simulink model "fix_Current_sync"  (R2025b)
settings: Solver=FixedStepAuto  StartTime=0.0  StopTime=20  FixedStep=0.001  RelTol=1e-3
values from neighbouring files (symbols this model uses):
  Dm = 1e-3    (= 0.001)    [motor_param.m]
  Ki_s = 0.041    [motor_param.m]
  Kp_s = 0.0014    [motor_param.m]
  Ld = 0.01    [motor_param.m]
  Lq = 0.02    [motor_param.m]
  p = 2    [motor_param.m]
  Phi = 0.1    [motor_param.m]
  Rs = 0.38    [motor_param.m]
libraries: fl_lib x50, nesl_utility x50, ee_lib x15, eeTransforms x10, slpidlib x5
(part 3 of 3)

== system fix_Current_sync/Subsystem5/Plant/MechSensor ==
  Ideal Rotational Motion Sensor : fl_lib/Mechanical/Mechanical Sensors/Ideal Rotational Motion Sensor  reference=foundation.enum.MeasurementReference.difference  acceleration_port=false  velocity_port=true  position_port=true  wrap_angle=simscape.enum.onoff.off  offset=0 rad
  Ideal Torque Sensor : fl_lib/Mechanical/Mechanical Sensors/Ideal Torque Sensor
  PS-Simulink Converter : nesl_utility/PS-Simulink Converter  PhysicalDomain=network_engine_domain  SubClassName=ps_output  LeftPortType=input  RightPortType=output  PseudoPeriodic=off  Frequencies=[]  VectorFormat=1-D array  Unit=1  AffineConversion=off
  PS-Simulink Converter1 : nesl_utility/PS-Simulink Converter  PhysicalDomain=network_engine_domain  SubClassName=ps_output  LeftPortType=input  RightPortType=output  PseudoPeriodic=off  Frequencies=[]  VectorFormat=1-D array  Unit=1  AffineConversion=off
  PS-Simulink Converter2 : nesl_utility/PS-Simulink Converter  PhysicalDomain=network_engine_domain  SubClassName=ps_output  LeftPortType=input  RightPortType=output  PseudoPeriodic=off  Frequencies=[]  VectorFormat=1-D array  Unit=1  AffineConversion=off
  R1 : PMIOPort  Side=Left
  C1 : PMIOPort  Port=2  Side=Left
  R2 : PMIOPort  Port=3  Side=Right
  C2 : PMIOPort  Port=4  Side=Right
  wm : Outport  VectorParamsAs1DForOutWhenUnconnected=off
  thm : Outport  Port=2  VectorParamsAs1DForOutWhenUnconnected=off
  Tm : Outport  Port=3  VectorParamsAs1DForOutWhenUnconnected=off
  wires:
  PS-Simulink Converter/1 -> thm/1
  PS-Simulink Converter1/1 -> Tm/1
  PS-Simulink Converter2/1 -> wm/1
  connections:
  Ideal Rotational Motion Sensor/RConn3 -- PS-Simulink Converter/LConn1
  Ideal Rotational Motion Sensor/RConn1 -- C2/RConn1 -- C1/RConn1
  Ideal Torque Sensor/LConn1 -- R1/RConn1
  Ideal Torque Sensor/RConn1 -- R2/RConn1 -- Ideal Rotational Motion Sensor/LConn1
  PS-Simulink Converter1/LConn1 -- Ideal Torque Sensor/RConn2
  Ideal Rotational Motion Sensor/RConn2 -- PS-Simulink Converter2/LConn1

== system fix_Current_sync/Subsystem1/Controller/DriverPeripherals/Break Algebraic Loop ==
  In1 : Inport
  Demux : Demux  Outputs=3
  Mux : Mux  Inputs=3
  Transfer Fcn : TransferFcn  Denominator=[1e-6 1]
  Transfer Fcn1 : TransferFcn  Denominator=[1e-6 1]
  Transfer Fcn2 : TransferFcn  Denominator=[1e-6 1]
  Out1 : Outport
  wires:
  In1/1 -> Demux/1
  Demux/1 -> Transfer Fcn/1
  Transfer Fcn/1 -> Mux/1
  Demux/2 -> Transfer Fcn1/1
  Transfer Fcn1/1 -> Mux/2
  Demux/3 -> Transfer Fcn2/1
  Transfer Fcn2/1 -> Mux/3
  Mux/1 -> Out1/1

== system fix_Current_sync/Subsystem1/Controller/FOC/CurrentController ==
  Iqref : Inport
  Id : Inport  Port=2
  Iq : Inport  Port=3
  we : Inport  Port=4
  Integrator : Integrator
  MATLAB Function : MATLAB Function  TreatAsAtomicUnit=on
  Scope : Scope
      settings: ActiveDisplayYMinimum=-0.021972241997855933  ActiveDisplayYMaximum=0.011100987286103392  DataLoggingVariableName=ScopeData15
  Scope1 : Scope
      settings: ActiveDisplayYMinimum=-15.558960108709503  ActiveDisplayYMaximum=12.807301262932642  DataLoggingVariableName=ScopeData10
  Scope2 : Scope
      settings: ActiveDisplayYMinimum=-2.450488291060998  ActiveDisplayYMaximum=2.3822321131147937  DataLoggingVariableName=ScopeData11
  Vdref : Outport  VectorParamsAs1DForOutWhenUnconnected=off
  Vqref : Outport  Port=2  VectorParamsAs1DForOutWhenUnconnected=off
  wires:
  Integrator/1 -> MATLAB Function/1(z_q)
  MATLAB Function/3(dz_q) -> Integrator/1
  MATLAB Function/4(e_q_bar) -> Scope/1
  MATLAB Function/1(Vq) -> Scope1/1, Vqref/1
  MATLAB Function/2(Vd) -> Scope2/1, Vdref/1
  we/1 -> MATLAB Function/5(we)
  Iqref/1 -> MATLAB Function/2(i_q_ref)
  Id/1 -> MATLAB Function/4(i_d)
  Iq/1 -> MATLAB Function/3(i_q)

== system fix_Current_sync/Subsystem1/Controller/FOC/VelocityController ==
  wmref : Inport
  wm : Inport  Port=2
  Gain : Gain  Gain=1/(3/2*p*Phi)
  PIDController : slpidlib/PID Controller  Controller=PI  Form=Parallel  TimeDomain=Continuous-time  UseExternalTs=off  SampleTime=-1  IntegratorMethod=Forward Euler  FilterMethod=Forward Euler  ControllerParametersSource=internal  P=Kp_s  I=Ki_s  UseKiTs=off  D=0  UseExternalDerivativeSource=off  N=100  UseFilter=on  TunerSelectOption=Transfer Function Based (PID Tuner App)  InitialConditionSource=internal  InitialConditionForIntegrator=0  InitialConditionForFilter=0  DifferentiatorICPrevScaledInput=0  ExternalReset=none  TrackingMode=off  Kt=1  LimitOutput=off  SatLimitsSource=internal  UpperSaturationLimit=inf  LowerSaturationLimit=-inf  LinearizeAsGain=on  AntiWindupMode=none  Kb=1  LimitIntegrator=off  UpperIntegratorSaturationLimit=inf  LowerIntegratorSaturationLimit=-inf  POutMin=[]  POutMax=[]  IOutMin=[]  IOutMax=[]  DOutMin=[]  DOutMax=[]  NOutMin=[]  NOutMax=[]  SumOutMin=[]  SumOutMax=[]  SaturationOutMin=[]  SaturationOutMax=[]  PParamMin=[]  PParamMax=[]  IParamMin=[]  IParamMax=[]  DParamMin=[]  DParamMax=[]  NParamMin=[]  NParamMax=[]  KbParamMin=[]  KbParamMax=[]  KtParamMin=[]  KtParamMax=[]  KbOutMin=[]  KbOutMax=[]  KtOutMin=[]  KtOutMax=[]  IntegratorOutMin=[]  IntegratorOutMax=[]  FilterOutMin=[]  FilterOutMax=[]  SumI1OutMin=[]  SumI1OutMax=[]  SumI2OutMin=[]  SumI2OutMax=[]  SumI3OutMin=[]  SumI3OutMax=[]  SumI4OutMin=[]  SumI4OutMax=[]  SumDOutMin=[]  SumDOutMax=[]  DifferentiatorOutMin=[]  DifferentiatorOutMax=[]  FilterDiffOutCoefMin=[]  FilterDiffOutCoefMax=[]  ReciprocalOutMin=[]  ReciprocalOutMax=[]  SumDenOutMin=[]  SumDenOutMax=[]  SumNumOutMin=[]  SumNumOutMax=[]  DivideOutMin=[]  DivideOutMax=[]  UdiffTsProdOutMin=[]  UdiffTsProdOutMax=[]  NTsProdOutMin=[]  NTsProdOutMax=[]  UintegralTsProdOutMin=[]  UintegralTsProdOutMax=[]  UngainTsProdOutMin=[]  UngainTsProdOutMax=[]  ClampingZeroOutDataTypeStr=Inherit: Inherit via back propagation  ClampingZeroOutMin=[]  ClampingZeroOutMax=[]  FilterDenConstantOutDataTypeStr=Inherit: Inherit via back propagation  FilterDenConstantOutMin=[]  FilterDenConstantOutMax=[]  PCopyOutDataTypeStr=Inherit: Inherit via back propagation  PCopyOutMin=[]  PCopyOutMax=[]  NCopyOutDataTypeStr=Inherit: Inherit via back propagation  NCopyOutMin=[]  NCopyOutMax=[]  IntegratorContinuousStateAttributes=''  IntegratorStateMustResolveToSignalObject=off  IntegratorRTWStateStorageClass=Auto  FilterContinuousStateAttributes=''  FilterStateMustResolveToSignalObject=off  FilterRTWStateStorageClass=Auto  ParallelPVariant=InternalParameters  IdealPVariant=Disabled  IVariant=InternalParameters  DVariant=Disabled  IntegratorVariant=Continuous  SatVariant=Disabled  AWVariant=Passthrough  PCopyVariant=Disabled  TRVariant=Disabled  FdbkBlocksVariant=Forward  IdealPFdbkVariant=Disabled  SatFdbkVariant=Disabled  DerivativeFilterVariant=Disabled  NVariant=Disabled  NCopyVariant=Disabled_SignalSpec  FilterICVariant=Disabled  IntegratorICVariant=InternalICs  ExternalResetVariant=Disabled  TRSumVariant=Passthrough  SumFdbkVariant=Disabled  SumVariant=Sum_PI  TsampFilterVariant=InternalTs  TsampNgainVariant=Passthrough  TsampIntegralVariant=Disabled_SignalSpec  ExternalSaturationOutDataTypeStr=Inherit: Same as second input  DerivativeSourceVariant=Disabled  PreIntVariant=InternalPreInt
  Sum : Sum  Inputs=|+-
  Iqref : Outport  VectorParamsAs1DForOutWhenUnconnected=off
  wires:
  Gain/1 -> Iqref/1
  wmref/1 -> Sum/1
  wm/1 -> Sum/2
  Sum/1 -> PIDController/1
  PIDController/1 -> Gain/1

== system fix_Current_sync/Subsystem1/Controller/FOC/abc2dq ==
  Iabc : Inport
  thetae : Inport  Port=2
  Demux1 : Demux  Outputs=3
  Park Transform : eeTransforms/Park Transform  AxisAlignment=D-axis  PowerInvariant=off
  Terminator : Terminator
  Id : Outport  VectorParamsAs1DForOutWhenUnconnected=off
  Iq : Outport  Port=2  VectorParamsAs1DForOutWhenUnconnected=off
  wires:
  Iabc/1 -> Park Transform/1
  thetae/1 -> Park Transform/2
  Demux1/3 -> Terminator/1
  Park Transform/1 -> Demux1/1
  Demux1/1 -> Id/1
  Demux1/2 -> Iq/1

== system fix_Current_sync/Subsystem1/Controller/FOC/dq2abc ==
  Vd : Inport
  Vq : Inport  Port=2
  thetae : Inport  Port=3
  Constant : Constant  Value=0
  Inverse Park Transform : eeTransforms/Inverse Park Transform  AxisAlignment=D-axis  PowerInvariant=off
  Mux : Mux  Inputs=3
  Vabc : Outport  VectorParamsAs1DForOutWhenUnconnected=off
  wires:
  thetae/1 -> Inverse Park Transform/2
  Constant/1 -> Mux/3
  Mux/1 -> Inverse Park Transform/1
  Vd/1 -> Mux/1
  Inverse Park Transform/1 -> Vabc/1
  Vq/1 -> Mux/2

== system fix_Current_sync/Subsystem1/Controller/FOC/thm2the ==
  thm : Inport
  Constant : Constant  Value=2*pi
  Mod : Math  Operator=mod  SignedPower=on
  PolePairs : Gain  Gain=p
  the : Outport  VectorParamsAs1DForOutWhenUnconnected=off
  wires:
  Constant/1 -> Mod/2
  PolePairs/1 -> Mod/1
  Mod/1 -> the/1
  thm/1 -> PolePairs/1

== system fix_Current_sync/Subsystem1/Controller/FOC/wm2we ==
  wm : Inport
  PolePairs : Gain  Gain=p
  we : Outport  VectorParamsAs1DForOutWhenUnconnected=off
  wires:
  wm/1 -> PolePairs/1
  PolePairs/1 -> we/1

== system fix_Current_sync/Subsystem2/Controller/DriverPeripherals/Break Algebraic Loop ==
  In1 : Inport
  Demux : Demux  Outputs=3
  Mux : Mux  Inputs=3
  Transfer Fcn : TransferFcn  Denominator=[1e-6 1]
  Transfer Fcn1 : TransferFcn  Denominator=[1e-6 1]
  Transfer Fcn2 : TransferFcn  Denominator=[1e-6 1]
  Out1 : Outport
  wires:
  In1/1 -> Demux/1
  Demux/1 -> Transfer Fcn/1
  Transfer Fcn/1 -> Mux/1
  Demux/2 -> Transfer Fcn1/1
  Transfer Fcn1/1 -> Mux/2
  Demux/3 -> Transfer Fcn2/1
  Transfer Fcn2/1 -> Mux/3
  Mux/1 -> Out1/1

== system fix_Current_sync/Subsystem2/Controller/FOC/CurrentController ==
  Iqref : Inport
  Id : Inport  Port=2
  Iq : Inport  Port=3
  we : Inport  Port=4
  Integrator : Integrator
  MATLAB Function : MATLAB Function  TreatAsAtomicUnit=on
  Scope : Scope
      settings: ActiveDisplayYMinimum=-0.021972241997855933  ActiveDisplayYMaximum=0.011100987286103392  DataLoggingVariableName=ScopeData9
  Vdref : Outport  VectorParamsAs1DForOutWhenUnconnected=off
  Vqref : Outport  Port=2  VectorParamsAs1DForOutWhenUnconnected=off
  wires:
  Id/1 -> MATLAB Function/4(i_d)
  MATLAB Function/3(dz_q) -> Integrator/1
  Integrator/1 -> MATLAB Function/1(z_q)
  MATLAB Function/1(Vq) -> Vqref/1
  MATLAB Function/2(Vd) -> Vdref/1
  we/1 -> MATLAB Function/5(we)
  Iqref/1 -> MATLAB Function/2(i_q_ref)
  Iq/1 -> MATLAB Function/3(i_q)
  MATLAB Function/4(e_q_bar) -> Scope/1

== system fix_Current_sync/Subsystem2/Controller/FOC/VelocityController ==
  wmref : Inport
  wm : Inport  Port=2
  Gain : Gain  Gain=1/(3/2*p*Phi)
  PIDController : slpidlib/PID Controller  Controller=PI  Form=Parallel  TimeDomain=Continuous-time  UseExternalTs=off  SampleTime=-1  IntegratorMethod=Forward Euler  FilterMethod=Forward Euler  ControllerParametersSource=internal  P=Kp_s  I=Ki_s  UseKiTs=off  D=0  UseExternalDerivativeSource=off  N=100  UseFilter=on  TunerSelectOption=Transfer Function Based (PID Tuner App)  InitialConditionSource=internal  InitialConditionForIntegrator=0  InitialConditionForFilter=0  DifferentiatorICPrevScaledInput=0  ExternalReset=none  TrackingMode=off  Kt=1  LimitOutput=off  SatLimitsSource=internal  UpperSaturationLimit=inf  LowerSaturationLimit=-inf  LinearizeAsGain=on  AntiWindupMode=none  Kb=1  LimitIntegrator=off  UpperIntegratorSaturationLimit=inf  LowerIntegratorSaturationLimit=-inf  POutMin=[]  POutMax=[]  IOutMin=[]  IOutMax=[]  DOutMin=[]  DOutMax=[]  NOutMin=[]  NOutMax=[]  SumOutMin=[]  SumOutMax=[]  SaturationOutMin=[]  SaturationOutMax=[]  PParamMin=[]  PParamMax=[]  IParamMin=[]  IParamMax=[]  DParamMin=[]  DParamMax=[]  NParamMin=[]  NParamMax=[]  KbParamMin=[]  KbParamMax=[]  KtParamMin=[]  KtParamMax=[]  KbOutMin=[]  KbOutMax=[]  KtOutMin=[]  KtOutMax=[]  IntegratorOutMin=[]  IntegratorOutMax=[]  FilterOutMin=[]  FilterOutMax=[]  SumI1OutMin=[]  SumI1OutMax=[]  SumI2OutMin=[]  SumI2OutMax=[]  SumI3OutMin=[]  SumI3OutMax=[]  SumI4OutMin=[]  SumI4OutMax=[]  SumDOutMin=[]  SumDOutMax=[]  DifferentiatorOutMin=[]  DifferentiatorOutMax=[]  FilterDiffOutCoefMin=[]  FilterDiffOutCoefMax=[]  ReciprocalOutMin=[]  ReciprocalOutMax=[]  SumDenOutMin=[]  SumDenOutMax=[]  SumNumOutMin=[]  SumNumOutMax=[]  DivideOutMin=[]  DivideOutMax=[]  UdiffTsProdOutMin=[]  UdiffTsProdOutMax=[]  NTsProdOutMin=[]  NTsProdOutMax=[]  UintegralTsProdOutMin=[]  UintegralTsProdOutMax=[]  UngainTsProdOutMin=[]  UngainTsProdOutMax=[]  ClampingZeroOutDataTypeStr=Inherit: Inherit via back propagation  ClampingZeroOutMin=[]  ClampingZeroOutMax=[]  FilterDenConstantOutDataTypeStr=Inherit: Inherit via back propagation  FilterDenConstantOutMin=[]  FilterDenConstantOutMax=[]  PCopyOutDataTypeStr=Inherit: Inherit via back propagation  PCopyOutMin=[]  PCopyOutMax=[]  NCopyOutDataTypeStr=Inherit: Inherit via back propagation  NCopyOutMin=[]  NCopyOutMax=[]  IntegratorContinuousStateAttributes=''  IntegratorStateMustResolveToSignalObject=off  IntegratorRTWStateStorageClass=Auto  FilterContinuousStateAttributes=''  FilterStateMustResolveToSignalObject=off  FilterRTWStateStorageClass=Auto  ParallelPVariant=InternalParameters  IdealPVariant=Disabled  IVariant=InternalParameters  DVariant=Disabled  IntegratorVariant=Continuous  SatVariant=Disabled  AWVariant=Passthrough  PCopyVariant=Disabled  TRVariant=Disabled  FdbkBlocksVariant=Forward  IdealPFdbkVariant=Disabled  SatFdbkVariant=Disabled  DerivativeFilterVariant=Disabled  NVariant=Disabled  NCopyVariant=Disabled_SignalSpec  FilterICVariant=Disabled  IntegratorICVariant=InternalICs  ExternalResetVariant=Disabled  TRSumVariant=Passthrough  SumFdbkVariant=Disabled  SumVariant=Sum_PI  TsampFilterVariant=InternalTs  TsampNgainVariant=Passthrough  TsampIntegralVariant=Disabled_SignalSpec  ExternalSaturationOutDataTypeStr=Inherit: Same as second input  DerivativeSourceVariant=Disabled  PreIntVariant=InternalPreInt
  Sum : Sum  Inputs=|+-
  Iqref : Outport  VectorParamsAs1DForOutWhenUnconnected=off
  wires:
  PIDController/1 -> Gain/1
  Gain/1 -> Iqref/1
  wmref/1 -> Sum/1
  Sum/1 -> PIDController/1
  wm/1 -> Sum/2

== system fix_Current_sync/Subsystem2/Controller/FOC/abc2dq ==
  Iabc : Inport
  thetae : Inport  Port=2
  Demux1 : Demux  Outputs=3
  Park Transform : eeTransforms/Park Transform  AxisAlignment=D-axis  PowerInvariant=off
  Terminator : Terminator
  Id : Outport  VectorParamsAs1DForOutWhenUnconnected=off
  Iq : Outport  Port=2  VectorParamsAs1DForOutWhenUnconnected=off
  wires:
  Iabc/1 -> Park Transform/1
  thetae/1 -> Park Transform/2
  Demux1/3 -> Terminator/1
  Park Transform/1 -> Demux1/1
  Demux1/1 -> Id/1
  Demux1/2 -> Iq/1

== system fix_Current_sync/Subsystem2/Controller/FOC/dq2abc ==
  Vd : Inport
  Vq : Inport  Port=2
  thetae : Inport  Port=3
  Constant : Constant  Value=0
  Inverse Park Transform : eeTransforms/Inverse Park Transform  AxisAlignment=D-axis  PowerInvariant=off
  Mux : Mux  Inputs=3
  Vabc : Outport  VectorParamsAs1DForOutWhenUnconnected=off
  wires:
  thetae/1 -> Inverse Park Transform/2
  Constant/1 -> Mux/3
  Mux/1 -> Inverse Park Transform/1
  Vd/1 -> Mux/1
  Inverse Park Transform/1 -> Vabc/1
  Vq/1 -> Mux/2

== system fix_Current_sync/Subsystem2/Controller/FOC/thm2the ==
  thm : Inport
  Constant : Constant  Value=2*pi
  Mod : Math  Operator=mod  SignedPower=on
  PolePairs : Gain  Gain=p
  the : Outport  VectorParamsAs1DForOutWhenUnconnected=off
  wires:
  Constant/1 -> Mod/2
  PolePairs/1 -> Mod/1
  Mod/1 -> the/1
  thm/1 -> PolePairs/1

== system fix_Current_sync/Subsystem2/Controller/FOC/wm2we ==
  wm : Inport
  PolePairs : Gain  Gain=p
  we : Outport  VectorParamsAs1DForOutWhenUnconnected=off
  wires:
  wm/1 -> PolePairs/1
  PolePairs/1 -> we/1

== system fix_Current_sync/Subsystem3/Controller/DriverPeripherals/Break Algebraic Loop ==
  In1 : Inport
  Demux : Demux  Outputs=3
  Mux : Mux  Inputs=3
  Transfer Fcn : TransferFcn  Denominator=[1e-6 1]
  Transfer Fcn1 : TransferFcn  Denominator=[1e-6 1]
  Transfer Fcn2 : TransferFcn  Denominator=[1e-6 1]
  Out1 : Outport
  wires:
  In1/1 -> Demux/1
  Demux/1 -> Transfer Fcn/1
  Transfer Fcn/1 -> Mux/1
  Demux/2 -> Transfer Fcn1/1
  Transfer Fcn1/1 -> Mux/2
  Demux/3 -> Transfer Fcn2/1
  Transfer Fcn2/1 -> Mux/3
  Mux/1 -> Out1/1

== system fix_Current_sync/Subsystem3/Controller/FOC/CurrentController ==
  Iqref : Inport
  Id : Inport  Port=2
  Iq : Inport  Port=3
  we : Inport  Port=4
  Integrator : Integrator
  MATLAB Function : MATLAB Function  TreatAsAtomicUnit=on
  Scope : Scope
      settings: ActiveDisplayYMinimum=-0.021972241997855933  ActiveDisplayYMaximum=0.011100987286103392  DataLoggingVariableName=ScopeData8
  Vdref : Outport  VectorParamsAs1DForOutWhenUnconnected=off
  Vqref : Outport  Port=2  VectorParamsAs1DForOutWhenUnconnected=off
  wires:
  Id/1 -> MATLAB Function/4(i_d)
  MATLAB Function/3(dz_q) -> Integrator/1
  Integrator/1 -> MATLAB Function/1(z_q)
  MATLAB Function/1(Vq) -> Vqref/1
  MATLAB Function/2(Vd) -> Vdref/1
  we/1 -> MATLAB Function/5(we)
  Iqref/1 -> MATLAB Function/2(i_q_ref)
  Iq/1 -> MATLAB Function/3(i_q)
  MATLAB Function/4(e_q_bar) -> Scope/1

== system fix_Current_sync/Subsystem3/Controller/FOC/VelocityController ==
  wmref : Inport
  wm : Inport  Port=2
  Gain : Gain  Gain=1/(3/2*p*Phi)
  PIDController : slpidlib/PID Controller  Controller=PI  Form=Parallel  TimeDomain=Continuous-time  UseExternalTs=off  SampleTime=-1  IntegratorMethod=Forward Euler  FilterMethod=Forward Euler  ControllerParametersSource=internal  P=Kp_s  I=Ki_s  UseKiTs=off  D=0  UseExternalDerivativeSource=off  N=100  UseFilter=on  TunerSelectOption=Transfer Function Based (PID Tuner App)  InitialConditionSource=internal  InitialConditionForIntegrator=0  InitialConditionForFilter=0  DifferentiatorICPrevScaledInput=0  ExternalReset=none  TrackingMode=off  Kt=1  LimitOutput=off  SatLimitsSource=internal  UpperSaturationLimit=inf  LowerSaturationLimit=-inf  LinearizeAsGain=on  AntiWindupMode=none  Kb=1  LimitIntegrator=off  UpperIntegratorSaturationLimit=inf  LowerIntegratorSaturationLimit=-inf  POutMin=[]  POutMax=[]  IOutMin=[]  IOutMax=[]  DOutMin=[]  DOutMax=[]  NOutMin=[]  NOutMax=[]  SumOutMin=[]  SumOutMax=[]  SaturationOutMin=[]  SaturationOutMax=[]  PParamMin=[]  PParamMax=[]  IParamMin=[]  IParamMax=[]  DParamMin=[]  DParamMax=[]  NParamMin=[]  NParamMax=[]  KbParamMin=[]  KbParamMax=[]  KtParamMin=[]  KtParamMax=[]  KbOutMin=[]  KbOutMax=[]  KtOutMin=[]  KtOutMax=[]  IntegratorOutMin=[]  IntegratorOutMax=[]  FilterOutMin=[]  FilterOutMax=[]  SumI1OutMin=[]  SumI1OutMax=[]  SumI2OutMin=[]  SumI2OutMax=[]  SumI3OutMin=[]  SumI3OutMax=[]  SumI4OutMin=[]  SumI4OutMax=[]  SumDOutMin=[]  SumDOutMax=[]  DifferentiatorOutMin=[]  DifferentiatorOutMax=[]  FilterDiffOutCoefMin=[]  FilterDiffOutCoefMax=[]  ReciprocalOutMin=[]  ReciprocalOutMax=[]  SumDenOutMin=[]  SumDenOutMax=[]  SumNumOutMin=[]  SumNumOutMax=[]  DivideOutMin=[]  DivideOutMax=[]  UdiffTsProdOutMin=[]  UdiffTsProdOutMax=[]  NTsProdOutMin=[]  NTsProdOutMax=[]  UintegralTsProdOutMin=[]  UintegralTsProdOutMax=[]  UngainTsProdOutMin=[]  UngainTsProdOutMax=[]  ClampingZeroOutDataTypeStr=Inherit: Inherit via back propagation  ClampingZeroOutMin=[]  ClampingZeroOutMax=[]  FilterDenConstantOutDataTypeStr=Inherit: Inherit via back propagation  FilterDenConstantOutMin=[]  FilterDenConstantOutMax=[]  PCopyOutDataTypeStr=Inherit: Inherit via back propagation  PCopyOutMin=[]  PCopyOutMax=[]  NCopyOutDataTypeStr=Inherit: Inherit via back propagation  NCopyOutMin=[]  NCopyOutMax=[]  IntegratorContinuousStateAttributes=''  IntegratorStateMustResolveToSignalObject=off  IntegratorRTWStateStorageClass=Auto  FilterContinuousStateAttributes=''  FilterStateMustResolveToSignalObject=off  FilterRTWStateStorageClass=Auto  ParallelPVariant=InternalParameters  IdealPVariant=Disabled  IVariant=InternalParameters  DVariant=Disabled  IntegratorVariant=Continuous  SatVariant=Disabled  AWVariant=Passthrough  PCopyVariant=Disabled  TRVariant=Disabled  FdbkBlocksVariant=Forward  IdealPFdbkVariant=Disabled  SatFdbkVariant=Disabled  DerivativeFilterVariant=Disabled  NVariant=Disabled  NCopyVariant=Disabled_SignalSpec  FilterICVariant=Disabled  IntegratorICVariant=InternalICs  ExternalResetVariant=Disabled  TRSumVariant=Passthrough  SumFdbkVariant=Disabled  SumVariant=Sum_PI  TsampFilterVariant=InternalTs  TsampNgainVariant=Passthrough  TsampIntegralVariant=Disabled_SignalSpec  ExternalSaturationOutDataTypeStr=Inherit: Same as second input  DerivativeSourceVariant=Disabled  PreIntVariant=InternalPreInt
  Sum : Sum  Inputs=|+-
  Iqref : Outport  VectorParamsAs1DForOutWhenUnconnected=off
  wires:
  PIDController/1 -> Gain/1
  Gain/1 -> Iqref/1
  wmref/1 -> Sum/1
  Sum/1 -> PIDController/1
  wm/1 -> Sum/2

== system fix_Current_sync/Subsystem3/Controller/FOC/abc2dq ==
  Iabc : Inport
  thetae : Inport  Port=2
  Demux1 : Demux  Outputs=3
  Park Transform : eeTransforms/Park Transform  AxisAlignment=D-axis  PowerInvariant=off
  Terminator : Terminator
  Id : Outport  VectorParamsAs1DForOutWhenUnconnected=off
  Iq : Outport  Port=2  VectorParamsAs1DForOutWhenUnconnected=off
  wires:
  Iabc/1 -> Park Transform/1
  thetae/1 -> Park Transform/2
  Demux1/3 -> Terminator/1
  Park Transform/1 -> Demux1/1
  Demux1/1 -> Id/1
  Demux1/2 -> Iq/1

== system fix_Current_sync/Subsystem3/Controller/FOC/dq2abc ==
  Vd : Inport
  Vq : Inport  Port=2
  thetae : Inport  Port=3
  Constant : Constant  Value=0
  Inverse Park Transform : eeTransforms/Inverse Park Transform  AxisAlignment=D-axis  PowerInvariant=off
  Mux : Mux  Inputs=3
  Vabc : Outport  VectorParamsAs1DForOutWhenUnconnected=off
  wires:
  thetae/1 -> Inverse Park Transform/2
  Constant/1 -> Mux/3
  Mux/1 -> Inverse Park Transform/1
  Vd/1 -> Mux/1
  Inverse Park Transform/1 -> Vabc/1
  Vq/1 -> Mux/2

== system fix_Current_sync/Subsystem3/Controller/FOC/thm2the ==
  thm : Inport
  Constant : Constant  Value=2*pi
  Mod : Math  Operator=mod  SignedPower=on
  PolePairs : Gain  Gain=p
  the : Outport  VectorParamsAs1DForOutWhenUnconnected=off
  wires:
  Constant/1 -> Mod/2
  PolePairs/1 -> Mod/1
  Mod/1 -> the/1
  thm/1 -> PolePairs/1

== system fix_Current_sync/Subsystem3/Controller/FOC/wm2we ==
  wm : Inport
  PolePairs : Gain  Gain=p
  we : Outport  VectorParamsAs1DForOutWhenUnconnected=off
  wires:
  wm/1 -> PolePairs/1
  PolePairs/1 -> we/1

== system fix_Current_sync/Subsystem4/Controller/DriverPeripherals/Break Algebraic Loop ==
  In1 : Inport
  Demux : Demux  Outputs=3
  Mux : Mux  Inputs=3
  Transfer Fcn : TransferFcn  Denominator=[1e-6 1]
  Transfer Fcn1 : TransferFcn  Denominator=[1e-6 1]
  Transfer Fcn2 : TransferFcn  Denominator=[1e-6 1]
  Out1 : Outport
  wires:
  In1/1 -> Demux/1
  Demux/1 -> Transfer Fcn/1
  Transfer Fcn/1 -> Mux/1
  Demux/2 -> Transfer Fcn1/1
  Transfer Fcn1/1 -> Mux/2
  Demux/3 -> Transfer Fcn2/1
  Transfer Fcn2/1 -> Mux/3
  Mux/1 -> Out1/1

== system fix_Current_sync/Subsystem4/Controller/FOC/CurrentController ==
  Iqref : Inport
  Id : Inport  Port=2
  Iq : Inport  Port=3
  we : Inport  Port=4
  Integrator : Integrator
  MATLAB Function : MATLAB Function  TreatAsAtomicUnit=on
  Scope : Scope
      settings: ActiveDisplayYMinimum=-0.021972241997855933  ActiveDisplayYMaximum=0.011100987286103392  DataLoggingVariableName=ScopeData7
  Vdref : Outport  VectorParamsAs1DForOutWhenUnconnected=off
  Vqref : Outport  Port=2  VectorParamsAs1DForOutWhenUnconnected=off
  wires:
  Id/1 -> MATLAB Function/4(i_d)
  MATLAB Function/3(dz_q) -> Integrator/1
  Integrator/1 -> MATLAB Function/1(z_q)
  MATLAB Function/1(Vq) -> Vqref/1
  MATLAB Function/2(Vd) -> Vdref/1
  we/1 -> MATLAB Function/5(we)
  Iqref/1 -> MATLAB Function/2(i_q_ref)
  Iq/1 -> MATLAB Function/3(i_q)
  MATLAB Function/4(e_q_bar) -> Scope/1

== system fix_Current_sync/Subsystem4/Controller/FOC/VelocityController ==
  wmref : Inport
  wm : Inport  Port=2
  Gain : Gain  Gain=1/(3/2*p*Phi)
  PIDController : slpidlib/PID Controller  Controller=PI  Form=Parallel  TimeDomain=Continuous-time  UseExternalTs=off  SampleTime=-1  IntegratorMethod=Forward Euler  FilterMethod=Forward Euler  ControllerParametersSource=internal  P=Kp_s  I=Ki_s  UseKiTs=off  D=0  UseExternalDerivativeSource=off  N=100  UseFilter=on  TunerSelectOption=Transfer Function Based (PID Tuner App)  InitialConditionSource=internal  InitialConditionForIntegrator=0  InitialConditionForFilter=0  DifferentiatorICPrevScaledInput=0  ExternalReset=none  TrackingMode=off  Kt=1  LimitOutput=off  SatLimitsSource=internal  UpperSaturationLimit=inf  LowerSaturationLimit=-inf  LinearizeAsGain=on  AntiWindupMode=none  Kb=1  LimitIntegrator=off  UpperIntegratorSaturationLimit=inf  LowerIntegratorSaturationLimit=-inf  POutMin=[]  POutMax=[]  IOutMin=[]  IOutMax=[]  DOutMin=[]  DOutMax=[]  NOutMin=[]  NOutMax=[]  SumOutMin=[]  SumOutMax=[]  SaturationOutMin=[]  SaturationOutMax=[]  PParamMin=[]  PParamMax=[]  IParamMin=[]  IParamMax=[]  DParamMin=[]  DParamMax=[]  NParamMin=[]  NParamMax=[]  KbParamMin=[]  KbParamMax=[]  KtParamMin=[]  KtParamMax=[]  KbOutMin=[]  KbOutMax=[]  KtOutMin=[]  KtOutMax=[]  IntegratorOutMin=[]  IntegratorOutMax=[]  FilterOutMin=[]  FilterOutMax=[]  SumI1OutMin=[]  SumI1OutMax=[]  SumI2OutMin=[]  SumI2OutMax=[]  SumI3OutMin=[]  SumI3OutMax=[]  SumI4OutMin=[]  SumI4OutMax=[]  SumDOutMin=[]  SumDOutMax=[]  DifferentiatorOutMin=[]  DifferentiatorOutMax=[]  FilterDiffOutCoefMin=[]  FilterDiffOutCoefMax=[]  ReciprocalOutMin=[]  ReciprocalOutMax=[]  SumDenOutMin=[]  SumDenOutMax=[]  SumNumOutMin=[]  SumNumOutMax=[]  DivideOutMin=[]  DivideOutMax=[]  UdiffTsProdOutMin=[]  UdiffTsProdOutMax=[]  NTsProdOutMin=[]  NTsProdOutMax=[]  UintegralTsProdOutMin=[]  UintegralTsProdOutMax=[]  UngainTsProdOutMin=[]  UngainTsProdOutMax=[]  ClampingZeroOutDataTypeStr=Inherit: Inherit via back propagation  ClampingZeroOutMin=[]  ClampingZeroOutMax=[]  FilterDenConstantOutDataTypeStr=Inherit: Inherit via back propagation  FilterDenConstantOutMin=[]  FilterDenConstantOutMax=[]  PCopyOutDataTypeStr=Inherit: Inherit via back propagation  PCopyOutMin=[]  PCopyOutMax=[]  NCopyOutDataTypeStr=Inherit: Inherit via back propagation  NCopyOutMin=[]  NCopyOutMax=[]  IntegratorContinuousStateAttributes=''  IntegratorStateMustResolveToSignalObject=off  IntegratorRTWStateStorageClass=Auto  FilterContinuousStateAttributes=''  FilterStateMustResolveToSignalObject=off  FilterRTWStateStorageClass=Auto  ParallelPVariant=InternalParameters  IdealPVariant=Disabled  IVariant=InternalParameters  DVariant=Disabled  IntegratorVariant=Continuous  SatVariant=Disabled  AWVariant=Passthrough  PCopyVariant=Disabled  TRVariant=Disabled  FdbkBlocksVariant=Forward  IdealPFdbkVariant=Disabled  SatFdbkVariant=Disabled  DerivativeFilterVariant=Disabled  NVariant=Disabled  NCopyVariant=Disabled_SignalSpec  FilterICVariant=Disabled  IntegratorICVariant=InternalICs  ExternalResetVariant=Disabled  TRSumVariant=Passthrough  SumFdbkVariant=Disabled  SumVariant=Sum_PI  TsampFilterVariant=InternalTs  TsampNgainVariant=Passthrough  TsampIntegralVariant=Disabled_SignalSpec  ExternalSaturationOutDataTypeStr=Inherit: Same as second input  DerivativeSourceVariant=Disabled  PreIntVariant=InternalPreInt
  Sum : Sum  Inputs=|+-
  Iqref : Outport  VectorParamsAs1DForOutWhenUnconnected=off
  wires:
  PIDController/1 -> Gain/1
  Gain/1 -> Iqref/1
  wmref/1 -> Sum/1
  Sum/1 -> PIDController/1
  wm/1 -> Sum/2

== system fix_Current_sync/Subsystem4/Controller/FOC/abc2dq ==
  Iabc : Inport
  thetae : Inport  Port=2
  Demux1 : Demux  Outputs=3
  Park Transform : eeTransforms/Park Transform  AxisAlignment=D-axis  PowerInvariant=off
  Terminator : Terminator
  Id : Outport  VectorParamsAs1DForOutWhenUnconnected=off
  Iq : Outport  Port=2  VectorParamsAs1DForOutWhenUnconnected=off
  wires:
  Iabc/1 -> Park Transform/1
  thetae/1 -> Park Transform/2
  Demux1/3 -> Terminator/1
  Park Transform/1 -> Demux1/1
  Demux1/1 -> Id/1
  Demux1/2 -> Iq/1

== system fix_Current_sync/Subsystem4/Controller/FOC/dq2abc ==
  Vd : Inport
  Vq : Inport  Port=2
  thetae : Inport  Port=3
  Constant : Constant  Value=0
  Inverse Park Transform : eeTransforms/Inverse Park Transform  AxisAlignment=D-axis  PowerInvariant=off
  Mux : Mux  Inputs=3
  Vabc : Outport  VectorParamsAs1DForOutWhenUnconnected=off
  wires:
  thetae/1 -> Inverse Park Transform/2
  Constant/1 -> Mux/3
  Mux/1 -> Inverse Park Transform/1
  Vd/1 -> Mux/1
  Inverse Park Transform/1 -> Vabc/1
  Vq/1 -> Mux/2

== system fix_Current_sync/Subsystem4/Controller/FOC/thm2the ==
  thm : Inport
  Constant : Constant  Value=2*pi
  Mod : Math  Operator=mod  SignedPower=on
  PolePairs : Gain  Gain=p
  the : Outport  VectorParamsAs1DForOutWhenUnconnected=off
  wires:
  Constant/1 -> Mod/2
  PolePairs/1 -> Mod/1
  Mod/1 -> the/1
  thm/1 -> PolePairs/1

== system fix_Current_sync/Subsystem4/Controller/FOC/wm2we ==
  wm : Inport
  PolePairs : Gain  Gain=p
  we : Outport  VectorParamsAs1DForOutWhenUnconnected=off
  wires:
  wm/1 -> PolePairs/1
  PolePairs/1 -> we/1

== system fix_Current_sync/Subsystem5/Controller/DriverPeripherals/Break Algebraic Loop ==
  In1 : Inport
  Demux : Demux  Outputs=3
  Mux : Mux  Inputs=3
  Transfer Fcn : TransferFcn  Denominator=[1e-6 1]
  Transfer Fcn1 : TransferFcn  Denominator=[1e-6 1]
  Transfer Fcn2 : TransferFcn  Denominator=[1e-6 1]
  Out1 : Outport
  wires:
  In1/1 -> Demux/1
  Demux/1 -> Transfer Fcn/1
  Transfer Fcn/1 -> Mux/1
  Demux/2 -> Transfer Fcn1/1
  Transfer Fcn1/1 -> Mux/2
  Demux/3 -> Transfer Fcn2/1
  Transfer Fcn2/1 -> Mux/3
  Mux/1 -> Out1/1

== system fix_Current_sync/Subsystem5/Controller/FOC/CurrentController ==
  Iqref : Inport
  Id : Inport  Port=2
  Iq : Inport  Port=3
  we : Inport  Port=4
  Integrator : Integrator
  MATLAB Function : MATLAB Function  TreatAsAtomicUnit=on
  Scope : Scope
      settings: ActiveDisplayYMinimum=-0.021972241997855933  ActiveDisplayYMaximum=0.011100987286103392  DataLoggingVariableName=ScopeData6
  Vdref : Outport  VectorParamsAs1DForOutWhenUnconnected=off
  Vqref : Outport  Port=2  VectorParamsAs1DForOutWhenUnconnected=off
  wires:
  Iqref/1 -> MATLAB Function/2(i_q_ref)
  we/1 -> MATLAB Function/5(we)
  Iq/1 -> MATLAB Function/3(i_q)
  MATLAB Function/4(e_q_bar) -> Scope/1
  Integrator/1 -> MATLAB Function/1(z_q)
  Id/1 -> MATLAB Function/4(i_d)
  MATLAB Function/3(dz_q) -> Integrator/1
  MATLAB Function/2(Vd) -> Vdref/1
  MATLAB Function/1(Vq) -> Vqref/1

== system fix_Current_sync/Subsystem5/Controller/FOC/VelocityController ==
  wmref : Inport
  wm : Inport  Port=2
  Gain : Gain  Gain=1/(3/2*p*Phi)
  PIDController : slpidlib/PID Controller  Controller=PI  Form=Parallel  TimeDomain=Continuous-time  UseExternalTs=off  SampleTime=-1  IntegratorMethod=Forward Euler  FilterMethod=Forward Euler  ControllerParametersSource=internal  P=Kp_s  I=Ki_s  UseKiTs=off  D=0  UseExternalDerivativeSource=off  N=100  UseFilter=on  TunerSelectOption=Transfer Function Based (PID Tuner App)  InitialConditionSource=internal  InitialConditionForIntegrator=0  InitialConditionForFilter=0  DifferentiatorICPrevScaledInput=0  ExternalReset=none  TrackingMode=off  Kt=1  LimitOutput=off  SatLimitsSource=internal  UpperSaturationLimit=inf  LowerSaturationLimit=-inf  LinearizeAsGain=on  AntiWindupMode=none  Kb=1  LimitIntegrator=off  UpperIntegratorSaturationLimit=inf  LowerIntegratorSaturationLimit=-inf  POutMin=[]  POutMax=[]  IOutMin=[]  IOutMax=[]  DOutMin=[]  DOutMax=[]  NOutMin=[]  NOutMax=[]  SumOutMin=[]  SumOutMax=[]  SaturationOutMin=[]  SaturationOutMax=[]  PParamMin=[]  PParamMax=[]  IParamMin=[]  IParamMax=[]  DParamMin=[]  DParamMax=[]  NParamMin=[]  NParamMax=[]  KbParamMin=[]  KbParamMax=[]  KtParamMin=[]  KtParamMax=[]  KbOutMin=[]  KbOutMax=[]  KtOutMin=[]  KtOutMax=[]  IntegratorOutMin=[]  IntegratorOutMax=[]  FilterOutMin=[]  FilterOutMax=[]  SumI1OutMin=[]  SumI1OutMax=[]  SumI2OutMin=[]  SumI2OutMax=[]  SumI3OutMin=[]  SumI3OutMax=[]  SumI4OutMin=[]  SumI4OutMax=[]  SumDOutMin=[]  SumDOutMax=[]  DifferentiatorOutMin=[]  DifferentiatorOutMax=[]  FilterDiffOutCoefMin=[]  FilterDiffOutCoefMax=[]  ReciprocalOutMin=[]  ReciprocalOutMax=[]  SumDenOutMin=[]  SumDenOutMax=[]  SumNumOutMin=[]  SumNumOutMax=[]  DivideOutMin=[]  DivideOutMax=[]  UdiffTsProdOutMin=[]  UdiffTsProdOutMax=[]  NTsProdOutMin=[]  NTsProdOutMax=[]  UintegralTsProdOutMin=[]  UintegralTsProdOutMax=[]  UngainTsProdOutMin=[]  UngainTsProdOutMax=[]  ClampingZeroOutDataTypeStr=Inherit: Inherit via back propagation  ClampingZeroOutMin=[]  ClampingZeroOutMax=[]  FilterDenConstantOutDataTypeStr=Inherit: Inherit via back propagation  FilterDenConstantOutMin=[]  FilterDenConstantOutMax=[]  PCopyOutDataTypeStr=Inherit: Inherit via back propagation  PCopyOutMin=[]  PCopyOutMax=[]  NCopyOutDataTypeStr=Inherit: Inherit via back propagation  NCopyOutMin=[]  NCopyOutMax=[]  IntegratorContinuousStateAttributes=''  IntegratorStateMustResolveToSignalObject=off  IntegratorRTWStateStorageClass=Auto  FilterContinuousStateAttributes=''  FilterStateMustResolveToSignalObject=off  FilterRTWStateStorageClass=Auto  ParallelPVariant=InternalParameters  IdealPVariant=Disabled  IVariant=InternalParameters  DVariant=Disabled  IntegratorVariant=Continuous  SatVariant=Disabled  AWVariant=Passthrough  PCopyVariant=Disabled  TRVariant=Disabled  FdbkBlocksVariant=Forward  IdealPFdbkVariant=Disabled  SatFdbkVariant=Disabled  DerivativeFilterVariant=Disabled  NVariant=Disabled  NCopyVariant=Disabled_SignalSpec  FilterICVariant=Disabled  IntegratorICVariant=InternalICs  ExternalResetVariant=Disabled  TRSumVariant=Passthrough  SumFdbkVariant=Disabled  SumVariant=Sum_PI  TsampFilterVariant=InternalTs  TsampNgainVariant=Passthrough  TsampIntegralVariant=Disabled_SignalSpec  ExternalSaturationOutDataTypeStr=Inherit: Same as second input  DerivativeSourceVariant=Disabled  PreIntVariant=InternalPreInt
  Sum : Sum  Inputs=|+-
  Iqref : Outport  VectorParamsAs1DForOutWhenUnconnected=off
  wires:
  PIDController/1 -> Gain/1
  Gain/1 -> Iqref/1
  wmref/1 -> Sum/1
  Sum/1 -> PIDController/1
  wm/1 -> Sum/2

== system fix_Current_sync/Subsystem5/Controller/FOC/abc2dq ==
  Iabc : Inport
  thetae : Inport  Port=2
  Demux1 : Demux  Outputs=3
  Park Transform : eeTransforms/Park Transform  AxisAlignment=D-axis  PowerInvariant=off
  Terminator : Terminator
  Id : Outport  VectorParamsAs1DForOutWhenUnconnected=off
  Iq : Outport  Port=2  VectorParamsAs1DForOutWhenUnconnected=off
  wires:
  Iabc/1 -> Park Transform/1
  thetae/1 -> Park Transform/2
  Demux1/3 -> Terminator/1
  Park Transform/1 -> Demux1/1
  Demux1/1 -> Id/1
  Demux1/2 -> Iq/1

== system fix_Current_sync/Subsystem5/Controller/FOC/dq2abc ==
  Vd : Inport
  Vq : Inport  Port=2
  thetae : Inport  Port=3
  Constant : Constant  Value=0
  Inverse Park Transform : eeTransforms/Inverse Park Transform  AxisAlignment=D-axis  PowerInvariant=off
  Mux : Mux  Inputs=3
  Vabc : Outport  VectorParamsAs1DForOutWhenUnconnected=off
  wires:
  thetae/1 -> Inverse Park Transform/2
  Constant/1 -> Mux/3
  Mux/1 -> Inverse Park Transform/1
  Vd/1 -> Mux/1
  Inverse Park Transform/1 -> Vabc/1
  Vq/1 -> Mux/2

== system fix_Current_sync/Subsystem5/Controller/FOC/thm2the ==
  thm : Inport
  Constant : Constant  Value=2*pi
  Mod : Math  Operator=mod  SignedPower=on
  PolePairs : Gain  Gain=p
  the : Outport  VectorParamsAs1DForOutWhenUnconnected=off
  wires:
  Constant/1 -> Mod/2
  PolePairs/1 -> Mod/1
  Mod/1 -> the/1
  thm/1 -> PolePairs/1

== system fix_Current_sync/Subsystem5/Controller/FOC/wm2we ==
  wm : Inport
  PolePairs : Gain  Gain=p
  we : Outport  VectorParamsAs1DForOutWhenUnconnected=off
  wires:
  wm/1 -> PolePairs/1
  PolePairs/1 -> we/1

== matlab function fix_Current_sync/Subsystem2/Controller/FOC/CurrentController/MATLAB Function ==
  data: z_q input; Vq output; i_q_ref input; i_q input; i_d input; we input; Vd output; dz_q output; e_q_bar output; Rs parameter; Ld parameter; Lq parameter; Phi parameter
function [Vq, Vd, dz_q, e_q_bar] = smc_ctrl(z_q, i_q_ref, i_q, i_d, we, Rs, Ld, Lq, Phi)
%#codegen
% ============================================================
%  PMSM 超螺旋滑模电流控制器
%  Rs, Ld, Lq, Phi, p 及滑模增益均由 Parameter 作用域提供
% ============================================================

%% ---------- 滑模参数 (仍然写死, 因为它们只属于控制器) ----------
r1  = 0.5;   r2  = 1.5;
rho1 = 0.5;  rho2 = 1.5;

k_q1 = -5000;  k_q2 = -4000;
k_d1 = -5000;  k_d2 = -4000;

lam_q1 = 50;   lam_q2 = 50;

%% ---------- 滑模面 ----------
e_q_bar = i_q - z_q;

%% ---------- 迭代部分的导数 (积分交给 Simulink) ----------
e_z  = z_q - i_q_ref;
dz_q = -lam_q1 * sig(e_z, rho1) - lam_q2 * sig(e_z, rho2);

%% ---------- u_q (非迭代) ----------
Vq = Lq * ( dz_q ...
             + k_q1 * sig(e_q_bar, r1) ...
             + k_q2 * sig(e_q_bar, r2) ) ...
      + Rs * z_q ...
      + Ld * we * i_d ...
      + we * Phi ;

%% ---------- u_d (非迭代) ----------
Vd = Ld * ( k_d1 * sig(i_d, r1) ...
             + k_d2 * sig(i_d, r2) ) ...
      + Rs * i_d ...
      + Lq * we * i_q;

end

function y = sig(x, r)
    y = abs(x)^r * sign(x);
end

== matlab function fix_Current_sync/Subsystem6/MATLAB Function ==
  data: theta0 input; omega_cmd output; theta_meas input; om_hat input
function omega_cmd  = Controller(theta0, theta_meas, om_hat)
%#codegen
% 输入:
%   theta0     - 领导者角度（标量）
%   theta_meas - 5x1 电机角度（编码器）
%   om_hat     - 5x1 前馈（观测器估计的领导者角速度）
%   v_f        - 5x1 低通滤波状态（来自 Integrator）
% 输出:
%   omega_cmd  - 5x1 未滤波控制器输出（仅记录/监控）
%   dv_f       - 5x1 滤波状态导数（送 Integrator）

n = 5;
L = 2*eye(n) - diag(ones(n-1,1),1) - diag(ones(n-1,1),-1);
B = diag([1, 0, 1, 0, 0]);

p1 = 0.75;  p2 = 1.5;
k1 = 5;    k2 = 5;

tau_f = 1e-2;   % ★ 低通时间常数

sig = @(x,a) sign(x).*abs(x).^a;
th0 = theta0(1);   % 强制标量

omega_cmd = zeros(n,1);
for i = 1:n
    ei = 0;
    for j = 1:n
        if i ~= j && L(i,j) ~= 0
            ei = ei + (-L(i,j))*(theta_meas(i) - theta_meas(j));
        end
    end
    if B(i,i) == 1
        ei = ei + (theta_meas(i) - th0);
    end
    omega_cmd(i) = min(max(om_hat(i) - k1*sig(ei,p1) - k2*sig(ei,p2),-50),50);
end


end

== matlab function fix_Current_sync/Subsystem6/MATLAB Function4 ==
  data: dth_hat output; dom_hat output; theta0 input; th_hat input; om_hat input
%% ObserverRHS
function [dth_hat, dom_hat] = ObserverRHS(theta0, th_hat, om_hat)
%#codegen
n = 5;
L = 2*eye(n) - diag(ones(n-1,1),1) - diag(ones(n-1,1),-1);
B = diag([1, 0, 1, 0, 0]);

a1 = 0.7;  a2 = 1.3;
a3 = 2*a1-1;  a4 = 2*a2-1;
c1 = 50;  c2 = 50;     % ★ 加大
c3 = 500; c4 = 500;    % ★ 加大

sig = @(x,a) sign(x).*abs(x).^a;

th0 = theta0(1);       % ★ 强制标量

e = zeros(n,1);
for i = 1:n
    ei = 0;
    for j = 1:n
        if i ~= j && L(i,j) ~= 0
            ei = ei + (-L(i,j))*(th_hat(i) - th_hat(j));
        end
    end
    if B(i,i) == 1
        ei = ei + (th_hat(i) - th0);
    end
    e(i) = ei;
end

dth_hat = om_hat - c1*sig(e,a1) - c2*sig(e,a2);
dom_hat =          - c3*sig(e,a3) - c4*sig(e,a4);
end

== matlab function fix_Current_sync/Subsystem5/Controller/FOC/CurrentController/MATLAB Function ==
  data: z_q input; Vq output; i_q_ref input; i_q input; i_d input; we input; Vd output; dz_q output; e_q_bar output; Rs parameter; Ld parameter; Lq parameter; Phi parameter
function [Vq, Vd, dz_q, e_q_bar] = smc_ctrl(z_q, i_q_ref, i_q, i_d, we, Rs, Ld, Lq, Phi)
%#codegen
% ============================================================
%  PMSM 超螺旋滑模电流控制器
%  Rs, Ld, Lq, Phi, p 及滑模增益均由 Parameter 作用域提供
% ============================================================

%% ---------- 滑模参数 (仍然写死, 因为它们只属于控制器) ----------
r1  = 0.5;   r2  = 1.5;
rho1 = 0.5;  rho2 = 1.5;

k_q1 = -5000;  k_q2 = -4000;
k_d1 = -5000;  k_d2 = -4000;

lam_q1 = 50;   lam_q2 = 50;

%% ---------- 滑模面 ----------
e_q_bar = i_q - z_q;

%% ---------- 迭代部分的导数 (积分交给 Simulink) ----------
e_z  = z_q - i_q_ref;
dz_q = -lam_q1 * sig(e_z, rho1) - lam_q2 * sig(e_z, rho2);

%% ---------- u_q (非迭代) ----------
Vq = Lq * ( dz_q ...
             + k_q1 * sig(e_q_bar, r1) ...
             + k_q2 * sig(e_q_bar, r2) ) ...
      + Rs * z_q ...
      + Ld * we * i_d ...
      + we * Phi ;

%% ---------- u_d (非迭代) ----------
Vd = Ld * ( k_d1 * sig(i_d, r1) ...
             + k_d2 * sig(i_d, r2) ) ...
      + Rs * i_d ...
      + Lq * we * i_q;

end

function y = sig(x, r)
    y = abs(x)^r * sign(x);
end

== matlab function fix_Current_sync/Subsystem1/Controller/FOC/CurrentController/MATLAB Function ==
  data: z_q input; Vq output; i_q_ref input; i_q input; i_d input; we input; Vd output; dz_q output; e_q_bar output; Rs parameter; Ld parameter; Lq parameter; Phi parameter
function [Vq, Vd, dz_q, e_q_bar] = smc_ctrl(z_q, i_q_ref, i_q, i_d, we, Rs, Ld, Lq, Phi)
%#codegen
% ============================================================
%  PMSM 超螺旋滑模电流控制器
%  Rs, Ld, Lq, Phi, p 及滑模增益均由 Parameter 作用域提供
% ============================================================

%% ---------- 滑模参数 (仍然写死, 因为它们只属于控制器) ----------
r1  = 0.5;   r2  = 1.5;
rho1 = 0.5;  rho2 = 1.5;

k_q1 = -5000;  k_q2 = -4000;
k_d1 = -5000;  k_d2 = -4000;

lam_q1 = 50;   lam_q2 = 50;

%% ---------- 滑模面 ----------
e_q_bar = i_q - z_q;

%% ---------- 迭代部分的导数 (积分交给 Simulink) ----------
e_z  = z_q - i_q_ref;
dz_q = -lam_q1 * sig(e_z, rho1) - lam_q2 * sig(e_z, rho2);

%% ---------- u_q (非迭代) ----------
Vq = Lq * ( dz_q ...
             + k_q1 * sig(e_q_bar, r1) ...
             + k_q2 * sig(e_q_bar, r2) ) ...
      + Rs * z_q ...
      + Ld * we * i_d ...
      + we * Phi ;

%% ---------- u_d (非迭代) ----------
Vd = Ld * ( k_d1 * sig(i_d, r1) ...
             + k_d2 * sig(i_d, r2) ) ...
      + Rs * i_d ...
      + Lq * we * i_q;

end

function y = sig(x, r)
    y = abs(x)^r * sign(x);
end

== matlab function fix_Current_sync/Subsystem4/Controller/FOC/CurrentController/MATLAB Function ==
  data: z_q input; Vq output; i_q_ref input; i_q input; i_d input; we input; Vd output; dz_q output; e_q_bar output; Rs parameter; Ld parameter; Lq parameter; Phi parameter
function [Vq, Vd, dz_q, e_q_bar] = smc_ctrl(z_q, i_q_ref, i_q, i_d, we, Rs, Ld, Lq, Phi)
%#codegen
% ============================================================
%  PMSM 超螺旋滑模电流控制器
%  Rs, Ld, Lq, Phi, p 及滑模增益均由 Parameter 作用域提供
% ============================================================

%% ---------- 滑模参数 (仍然写死, 因为它们只属于控制器) ----------
r1  = 0.5;   r2  = 1.5;
rho1 = 0.5;  rho2 = 1.5;

k_q1 = -5000;  k_q2 = -4000;
k_d1 = -5000;  k_d2 = -4000;

lam_q1 = 50;   lam_q2 = 50;

%% ---------- 滑模面 ----------
e_q_bar = i_q - z_q;

%% ---------- 迭代部分的导数 (积分交给 Simulink) ----------
e_z  = z_q - i_q_ref;
dz_q = -lam_q1 * sig(e_z, rho1) - lam_q2 * sig(e_z, rho2);

%% ---------- u_q (非迭代) ----------
Vq = Lq * ( dz_q ...
             + k_q1 * sig(e_q_bar, r1) ...
             + k_q2 * sig(e_q_bar, r2) ) ...
      + Rs * z_q ...
      + Ld * we * i_d ...
      + we * Phi ;

%% ---------- u_d (非迭代) ----------
Vd = Ld * ( k_d1 * sig(i_d, r1) ...
             + k_d2 * sig(i_d, r2) ) ...
      + Rs * i_d ...
      + Lq * we * i_q;

end

function y = sig(x, r)
    y = abs(x)^r * sign(x);
end

== matlab function fix_Current_sync/Subsystem3/Controller/FOC/CurrentController/MATLAB Function ==
  data: z_q input; Vq output; i_q_ref input; i_q input; i_d input; we input; Vd output; dz_q output; e_q_bar output; Rs parameter; Ld parameter; Lq parameter; Phi parameter
function [Vq, Vd, dz_q, e_q_bar] = smc_ctrl(z_q, i_q_ref, i_q, i_d, we, Rs, Ld, Lq, Phi)
%#codegen
% ============================================================
%  PMSM 超螺旋滑模电流控制器
%  Rs, Ld, Lq, Phi, p 及滑模增益均由 Parameter 作用域提供
% ============================================================

%% ---------- 滑模参数 (仍然写死, 因为它们只属于控制器) ----------
r1  = 0.5;   r2  = 1.5;
rho1 = 0.5;  rho2 = 1.5;

k_q1 = -5000;  k_q2 = -4000;
k_d1 = -5000;  k_d2 = -4000;

lam_q1 = 50;   lam_q2 = 50;

%% ---------- 滑模面 ----------
e_q_bar = i_q - z_q;

%% ---------- 迭代部分的导数 (积分交给 Simulink) ----------
e_z  = z_q - i_q_ref;
dz_q = -lam_q1 * sig(e_z, rho1) - lam_q2 * sig(e_z, rho2);

%% ---------- u_q (非迭代) ----------
Vq = Lq * ( dz_q ...
             + k_q1 * sig(e_q_bar, r1) ...
             + k_q2 * sig(e_q_bar, r2) ) ...
      + Rs * z_q ...
      + Ld * we * i_d ...
      + we * Phi ;

%% ---------- u_d (非迭代) ----------
Vd = Ld * ( k_d1 * sig(i_d, r1) ...
             + k_d2 * sig(i_d, r2) ) ...
      + Rs * i_d ...
      + Lq * we * i_q;

end

function y = sig(x, r)
    y = abs(x)^r * sign(x);
end
